simulink model "modelo_1_linear"  (R2026a)
settings: Solver=ode45  StopTime=8
libraries: cstblocks_lti x3

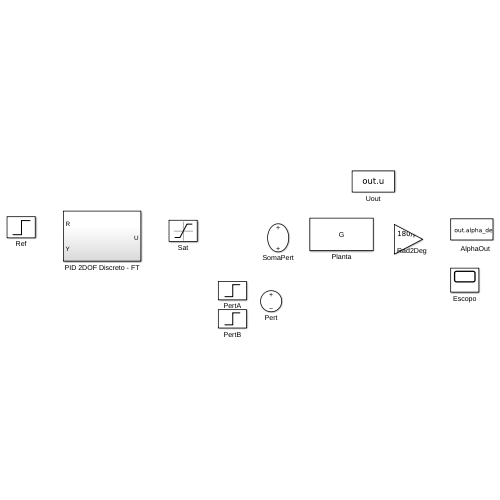
[thumbnail: Simulink's stored preview of the top-level diagram]
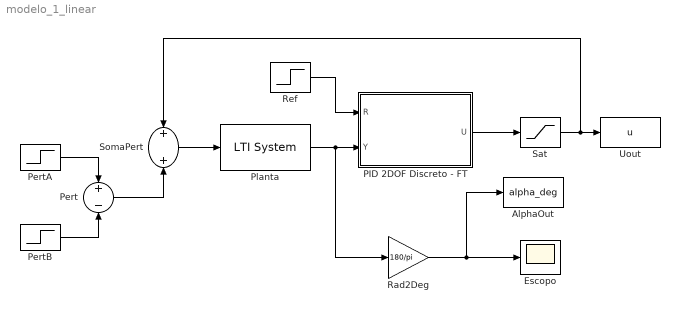
== system modelo_1_linear ==
  AlphaOut : ToWorkspace  VariableName=alpha_deg  SaveFormat=Timeseries  SampleTime=-1
  Escopo : Scope
  PID 2DOF Discreto - FT : Subsystem
  Pert : Sum  Inputs=+-
  PertA : Step  Time=2  FinalValue=60  SampleTime=0
  PertB : Step  Time=2.3  FinalValue=60  SampleTime=0
  Planta : cstblocks_lti/LTI System  sys=G  IC=[]  PadeOrder=0
      settings: LibrarySourceBlock=cstblocks/LTI System
  Rad2Deg : Gain  Gain=180/pi
  Ref : Step  Time=0  FinalValue=0  SampleTime=0
  Sat : Saturate  UpperLimit=255  LowerLimit=-255
  SomaPert : Sum
  Uout : ToWorkspace  VariableName=u  SaveFormat=Timeseries  SampleTime=-1
  wires:
  Sat/1 -> Uout/1, SomaPert/1
  Rad2Deg/1 -> Escopo/1, AlphaOut/1
  PID 2DOF Discreto - FT/1(U) -> Sat/1
  Ref/1 -> PID 2DOF Discreto - FT/1(R)
  SomaPert/1 -> Planta/1
  Pert/1 -> SomaPert/2
  Planta/1 -> PID 2DOF Discreto - FT/2(Y), Rad2Deg/1
  PertB/1 -> Pert/2
  PertA/1 -> Pert/1

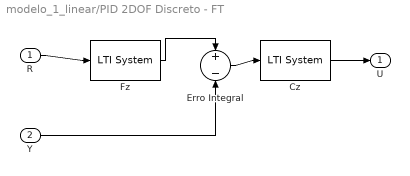
== system modelo_1_linear/PID 2DOF Discreto - FT ==
  R : Inport
  Y : Inport  Port=2
  Cz : cstblocks_lti/LTI System  sys=Cz  IC=[]  PadeOrder=0
      settings: LibrarySourceBlock=cstblocks/LTI System
  Erro Integral : Sum  Inputs=+-
  Fz : cstblocks_lti/LTI System  sys=Fz  IC=[]  PadeOrder=0
      settings: LibrarySourceBlock=cstblocks/LTI System
  U : Outport
  wires:
  R/1 -> Fz/1
  Fz/1 -> Erro Integral/1
  Y/1 -> Erro Integral/2
  Erro Integral/1 -> Cz/1
  Cz/1 -> U/1
